simulink model "HS_switchable_1_and_2"  (Simulink 8.6)
settings: Solver=ode3  SolverMode=SingleTasking  StartTime=0.0  StopTime=100000  FixedStep=dtModelRate  RelTol=1e-3
InitFcn:
  | dtModelRate = 0.001
settings Model: Creator=Craig  LastModifiedBy=Craig
settings SolverCC: EnableConcurrentExecution=on  ConcurrentTasks=on  PositivePriorityOrder=on  AutoInsertRateTranBlk=on
settings DataIOCC: LimitDataPoints=off  SaveFormat=Dataset  SignalLoggingSaveFormat=Dataset  SaveOutput=off  DSMLogging=off  SaveTime=off
settings OptimizationCC: BlockReduction=off  OptimizeBlockIOStorage=off  ExpressionDepthLimit=128  SimCompilerOptimization=on
settings DebuggingCC: UnderspecifiedInitializationDetection=Simplified  MergeDetectMultiDrivingBlocksExec=error  SolverPrmCheckMsg=none  TasksWithSamePriorityMsg=none  FcnCallInpInsideContextMsg=EnableAllAsError  AllowSymbolicDim=on  ModelReferenceSymbolNameMessage=none  StateNameClashWarn=none  BusNameAdapt=ErrorWithoutRepair  SFUnexpectedBacktrackingDiag=error  SFNoUnconditionalDefaultTransitionDiag=error
settings HardwareCC: ProdBitPerLong=64  ProdBitPerPointer=64  ProdLargestAtomicFloat=Float  ProdIntDivRoundTo=Zero  ProdEndianess=LittleEndian  ProdWordSize=64  ProdLongLongMode=on  ProdHWDeviceType=Intel->x86-64 (Linux 64)
settings ModelReferenceCC: PropagateSignalLabelsOutOfModel=on
settings SFSimCC: SimUseLocalCustomCode=on
settings RTWCC: Description=Simulink Real-Time  SystemTargetFile=slrealtime.tlc  TemplateMakefile=slrealtime_default_tmf  RTWUseLocalCustomCode=on  CustomLibrary=libCanopyDiL.a libCanopyDiLSFunContentsInline.a libgtest.a libgtest_main.a liblinSolve.a libePhyseNet_speedgoat.a libmsgpackc.a libpanthera_base-static.a  Toolchain=Simulink Real-Time Toolchain  BuildConfiguration=Faster Runs  CodeExecutionProfiling=on  TargetLang=C++
settings SimulinkRealTimeTargetCC: ERTMultiwordTypeDef=System defined  ExtMode=off  SLRTForcePollingMode=on
settings ConfigComp: CovMetricSettings=dwe  CovSaveCumulativeToWorkspaceVar=off  CovSaveSingleToWorkspaceVar=off  CovExternalEMLEnable=on

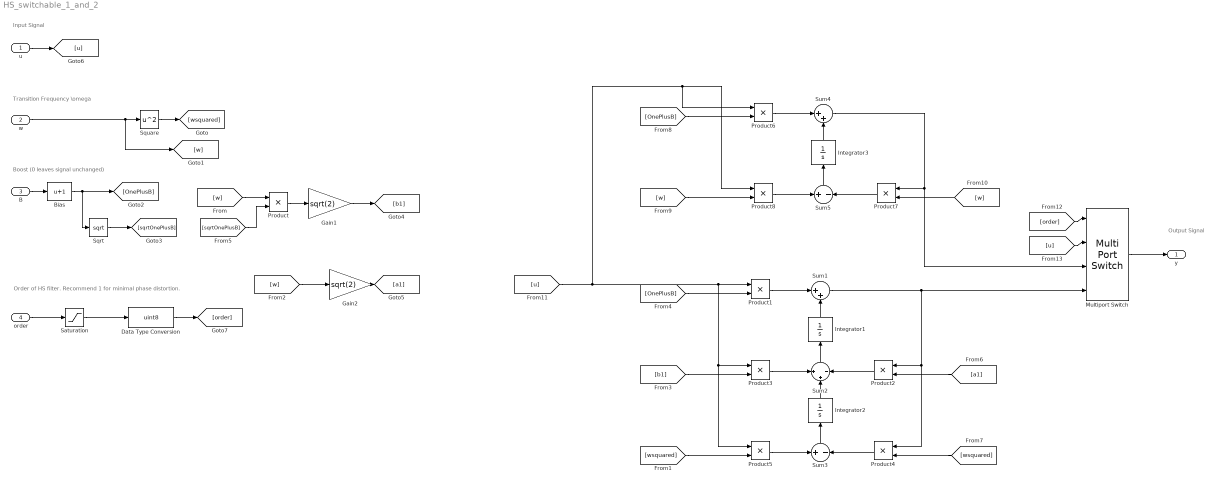
== system HS_switchable_1_and_2 ==
  note: Input Signal
  note: Transition Frequency \omega
  note: Boost (0 leaves signal unchanged)
  note: Order of HS filter. Recommend 1 for minimal phase distortion.
  note: Output Signal
  u : Inport
  w : Inport  Port=2
  B : Inport  Port=3
  order : Inport  Port=4
  Bias : Bias  Bias=1
  Data Type Conversion : DataTypeConversion  OutDataTypeStr=uint8
  Gain1 : Gain  Gain=sqrt(2)
  Gain2 : Gain  Gain=sqrt(2)
  Integrator1 : Integrator
  Integrator2 : Integrator
  Integrator3 : Integrator
  Multiport Switch : MultiPortSwitch  DataPortOrder=Zero-based contiguous  zeroidx=on
  Product{,1..8} (9 alike) : Product
  Saturation : Saturate  UpperLimit=2  LowerLimit=0
  Sqrt : Sqrt  SaturateOnIntegerOverflow=on
  Square : Math  Operator=square  SaturateOnIntegerOverflow=on
  Sum1 : Sum  Inputs=|++
  Sum2 : Sum  Inputs=+|+|-
  Sum3 : Sum  Inputs=+|-
  Sum4 : Sum  Inputs=|++
  Sum5 : Sum  Inputs=+|-
  y : Outport
  wires:
  [wsquared] -> Product5/2
  Product4/1 -> Sum3/2
  Integrator2/1 -> Sum2/2
  [b1] -> Product3/2
  [OnePlusB] -> Product1/2
  Product5/1 -> Sum3/1
  [wsquared] -> Product4/2
  Sum1/1 -> Product2/1, Product4/1, Multiport Switch/4
  [a1] -> Product2/2
  Integrator1/1 -> Sum1/2
  Product3/1 -> Sum2/1
  Product1/1 -> Sum1/1
  Product2/1 -> Sum2/3
  Sum2/1 -> Integrator1/1
  Sum3/1 -> Integrator2/1
  B/1 -> Bias/1
  w/1 -> [w], Square/1
  Square/1 -> [wsquared]
  Bias/1 -> Sqrt/1, [OnePlusB]
  Sqrt/1 -> [sqrtOnePlusB]
  Product/1 -> Gain1/1
  [w] -> Product/1
  [sqrtOnePlusB] -> Product/2
  Gain1/1 -> [b1]
  [w] -> Gain2/1
  Gain2/1 -> [a1]
  Multiport Switch/1 -> y/1
  [w] -> Product8/2
  Sum4/1 -> Multiport Switch/3, Product7/1
  Product7/1 -> Sum5/2
  Product6/1 -> Sum4/1
  [OnePlusB] -> Product6/2
  Sum5/1 -> Integrator3/1
  Integrator3/1 -> Sum4/2
  [u] -> Product6/1, Product8/1, Product3/1, Product5/1, Product1/1
  Product8/1 -> Sum5/1
  [w] -> Product7/2
  u/1 -> [u]
  order/1 -> Saturation/1
  Saturation/1 -> Data Type Conversion/1
  Data Type Conversion/1 -> [order]
  [order] -> Multiport Switch/1
  [u] -> Multiport Switch/2
